simulink model "lab7_simulink"  (R2021b)
settings: Solver=VariableStepAuto  StartTime=0.0  StopTime=24.0  RelTol=1e-3
settings Model: Creator=13676840  LastModifiedBy=13676840

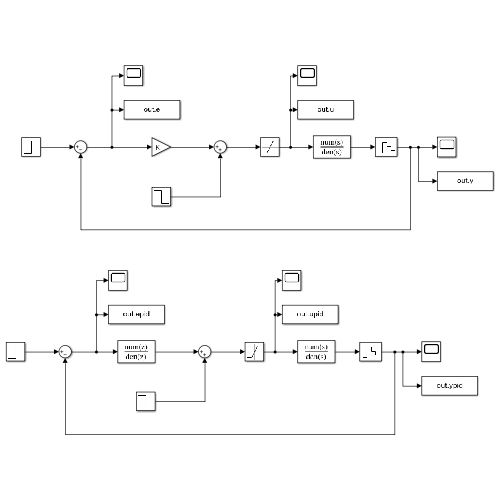
[thumbnail: Simulink's stored preview of the top-level diagram]
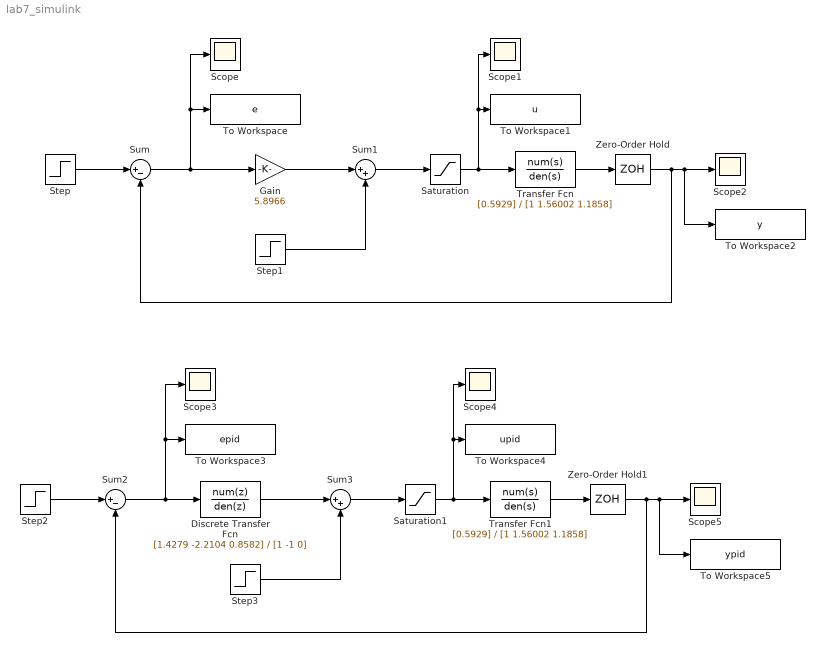
== system lab7_simulink ==
  Discrete Transfer Fcn : DiscreteTransferFcn  Numerator=[1.4279 -2.2104 0.8582]  Denominator=[1 -1 0]
  Gain : Gain  Gain=5.8966
  Saturation : Saturate  UpperLimit=10  LowerLimit=-10
  Saturation1 : Saturate  UpperLimit=10  LowerLimit=-10
  Scope{,1..5} (6 alike) : Scope
  Step : Step  Time=0  After=1.17  SampleTime=0
  Step1 : Step  Time=12  After=-0.15  SampleTime=0
  Step2 : Step  Time=0  After=1.17  SampleTime=0
  Step3 : Step  Time=12  After=-0.15  SampleTime=0
  Sum : Sum  Inputs=|+-
  Sum1 : Sum  Inputs=|++
  Sum2 : Sum  Inputs=|+-
  Sum3 : Sum  Inputs=|++
  To Workspace : ToWorkspace  VariableName=e  SaveFormat=Timeseries  SampleTime=-1
  To Workspace1 : ToWorkspace  VariableName=u  SaveFormat=Timeseries  SampleTime=-1
  To Workspace2 : ToWorkspace  VariableName=y  SaveFormat=Timeseries  SampleTime=-1
  To Workspace3 : ToWorkspace  VariableName=epid  SaveFormat=Timeseries  SampleTime=-1
  To Workspace4 : ToWorkspace  VariableName=upid  SaveFormat=Timeseries  SampleTime=-1
  To Workspace5 : ToWorkspace  VariableName=ypid  SaveFormat=Timeseries  SampleTime=-1
  Transfer Fcn : TransferFcn  Numerator=[0.5929]  Denominator=[1 1.56002 1.1858]
  Transfer Fcn1 : TransferFcn  Numerator=[0.5929]  Denominator=[1 1.56002 1.1858]
  Zero-Order Hold : ZeroOrderHold  SampleTime=0.2241
  Zero-Order Hold1 : ZeroOrderHold  SampleTime=0.2241
  wires:
  Step/1 -> Sum/1
  Sum/1 -> To Workspace/1, Scope/1, Gain/1
  Gain/1 -> Sum1/1
  Sum1/1 -> Saturation/1
  Saturation/1 -> To Workspace1/1, Scope1/1, Transfer Fcn/1
  Transfer Fcn/1 -> Zero-Order Hold/1
  Zero-Order Hold/1 -> Sum/2, To Workspace2/1, Scope2/1
  Step1/1 -> Sum1/2
  Transfer Fcn1/1 -> Zero-Order Hold1/1
  Saturation1/1 -> To Workspace4/1, Scope4/1, Transfer Fcn1/1
  Sum2/1 -> Discrete Transfer Fcn/1, To Workspace3/1, Scope3/1
  Zero-Order Hold1/1 -> Sum2/2, To Workspace5/1, Scope5/1
  Sum3/1 -> Saturation1/1
  Step2/1 -> Sum2/1
  Step3/1 -> Sum3/2
  Discrete Transfer Fcn/1 -> Sum3/1
